simulink model "Pulse_Radar"  (R2026a)
settings: Solver=FixedStepDiscrete  StopTime=T_stop
values from neighbouring files (symbols this model uses):
  alpha = N_train * (Pfa^(-1/N_train) - 1)    (= 13.9867223149)    [centroid_2d.m]    (also in init.m = 17.2776488339)
  cfar_delay = (N_train/2) + (N_guard/2)    (= 116)    [init.m]
  cfar_window = [ones(1, N_train/2), zeros(1, N_guard + 1), ones(1, N_train/2)] / N_train    [init.m]
  current_seed = randi(100000)    [centroid_test.m]    (also in multi_target_test.m; os_cfar_test.m = seeds(k); run_monte_carlo.m; velocity_test.m = 12345)
  doppler_window = hamming(N_cpi)'    [init.m]
  drop_threshold_delay = 8    [init.m]
  fd = (2 * target_velocity) / lambda    [init.m]    (also in velocity_test.m)
  H_delay = exp(-1j*2*pi*k_idx*N_delay/N)    [init.m]
  hardware_delay_samples = matched_filter_delay + cfar_delay + drop_threshold_delay    [init.m]
  lambda = c / fc    (= 0.03)    [init.m]
  MTI_delay = N_PRI    [init.m]
  N_cpi = 16    [init.m]
  N_PRI = round(PRI / Ts)    [init.m]
  N_tau_p = round(tau_p / Ts)    [init.m]
  noise_variance_IQ = Pn / 2    (= 3.99251989225e-15)    [init.m]
  radar_const = (Pt * G^2 * lambda^2) ./ (((4*pi)^3) * (range.^4) * L)    [init.m]
  range = [20e3 40e3 70e3]    [init.m]
  range_per_sample = (c * Ts) / 2    (= 150)    [init.m]
  T_stop = N_cpi * PRI    (= 0.016)    [init.m]
  target_rcs = [1 1 1]    [init.m]
  Ts = 1e-6    (= 1e-06)    [init.m]
undefined symbols (not defined in the file or in its folder): dspblkCoreblockFVToolHelper, gcbh, get, jet, magnitude, Radix
libraries: dspxfrm3 x3, dspobslib x2, simulink x1
settings Model: Creator=daksh  LastModifiedBy=daksh

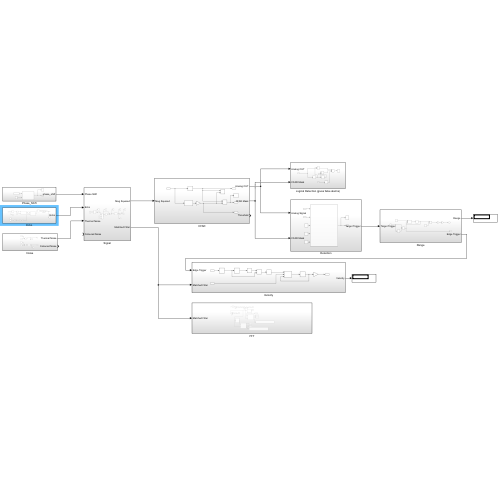
[thumbnail: Simulink's stored preview of the top-level diagram]
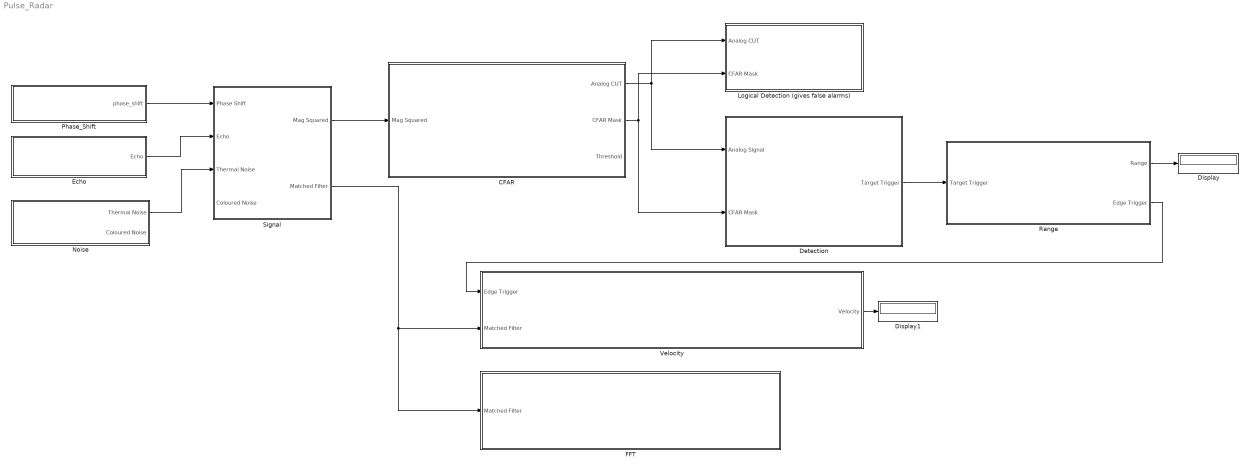
== system Pulse_Radar ==
  CFAR : Subsystem
  Detection : Subsystem
  Display : Display
  Display1 : Display
  Echo : Subsystem
  FFT : Subsystem
  Logical Detection (gives false alarms) : Subsystem
  Noise : Subsystem
  Phase_Shift : Subsystem
  Range : Subsystem
  Signal : Subsystem
  Velocity : Subsystem
  wires:
  Range/1(Range) -> Display/1
  Velocity/1(Velocity) -> Display1/1
  Noise/1(Thermal Noise) -> Signal/3(Thermal Noise)
  CFAR/1(Analog CUT) -> Logical Detection (gives false alarms)/1(Analog CUT), Detection/1(Analog Signal)
  CFAR/2(CFAR Mask) -> Detection/2(CFAR Mask), Logical Detection (gives false alarms)/2(CFAR Mask)
  Detection/1(Target Trigger) -> Range/1(Target Trigger)
  Range/2(Edge Trigger) -> Velocity/1(Edge Trigger)
  Echo/1(Echo) -> Signal/2(Echo)
  Phase_Shift/1(phase_shift) -> Signal/1(Phase Shift)
  Signal/1(Mag Squared) -> CFAR/1(Mag Squared)
  Signal/2(Matched Filter) -> FFT/1(Matched Filter), Velocity/2(Matched Filter)

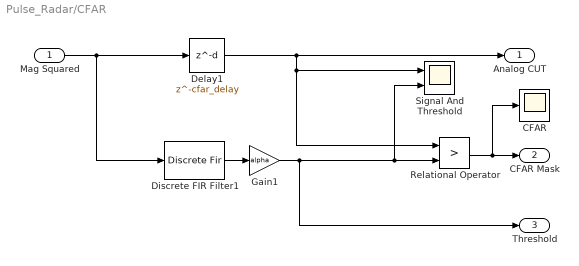
== system Pulse_Radar/CFAR ==
  Mag Squared : Inport
  CFAR : Scope
      settings: ActiveDisplayYMinimum=-1  ActiveDisplayYMaximum=1  DataLoggingVariableName=ScopeData10
  Delay1 : Delay  DelayLength=cfar_delay
  Discrete FIR Filter1 : DiscreteFir  LoadFcn=dspblkCoreblockFVToolHelper(gcbh,'load');  Coefficients=cfar_window
      settings: CopyFcn=dspblkCoreblockFVToolHelper(gcbh,'copy');  DeleteFcn=dspblkCoreblockFVToolHelper(gcbh,'close');  ModelCloseFcn=dspblkCoreblockFVToolHelper(gcbh,'close');  PreSaveFcn=dspblkCoreblockFVToolHelper(gcbh,'presave');  PostSaveFcn=dspblkCoreblockFVToolHelper(gcbh,'postsave');  CloseFcn=dspblkCoreblockFVToolHelper(gcbh,'close');
  Gain1 : Gain  Gain=alpha
  Relational Operator : RelationalOperator  Operator=>  OutDataTypeStr=boolean  RndMeth=Simplest  InputSameDT=off
  Signal And Threshold : Scope  NumInputPorts=2
      settings: ActiveDisplayYMinimum=-3.5614234572885921E-9  ActiveDisplayYMaximum=3.2052811115597338E-8  DataLoggingVariableName=ScopeData9
  Analog CUT : Outport
  CFAR Mask : Outport  Port=2
  Threshold : Outport  Port=3
  wires:
  Gain1/1 -> Signal And Threshold/2, Relational Operator/2, Threshold/1
  Discrete FIR Filter1/1 -> Gain1/1
  Mag Squared/1 -> Discrete FIR Filter1/1, Delay1/1
  Relational Operator/1 -> CFAR/1, CFAR Mask/1
  Delay1/1 -> Relational Operator/1, Signal And Threshold/1, Analog CUT/1

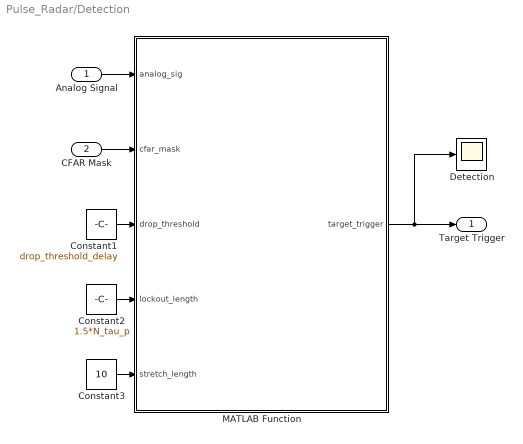
== system Pulse_Radar/Detection ==
  Analog Signal : Inport
  CFAR Mask : Inport  Port=2
  Constant1 : Constant  Value=drop_threshold_delay
  Constant2 : Constant  Value=1.5*N_tau_p
  Constant3 : Constant  Value=10
  Detection : Scope
      settings: ActiveDisplayYMinimum=-1  ActiveDisplayYMaximum=1  DataLoggingVariableName=ScopeData9
  MATLAB Function : MATLAB Function  TreatAsAtomicUnit=on
  Target Trigger : Outport
  wires:
  Constant3/1 -> MATLAB Function/5(stretch_length)
  Constant1/1 -> MATLAB Function/3(drop_threshold)
  Constant2/1 -> MATLAB Function/4(lockout_length)
  Analog Signal/1 -> MATLAB Function/1(analog_sig)
  CFAR Mask/1 -> MATLAB Function/2(cfar_mask)
  MATLAB Function/1(target_trigger) -> Detection/1, Target Trigger/1

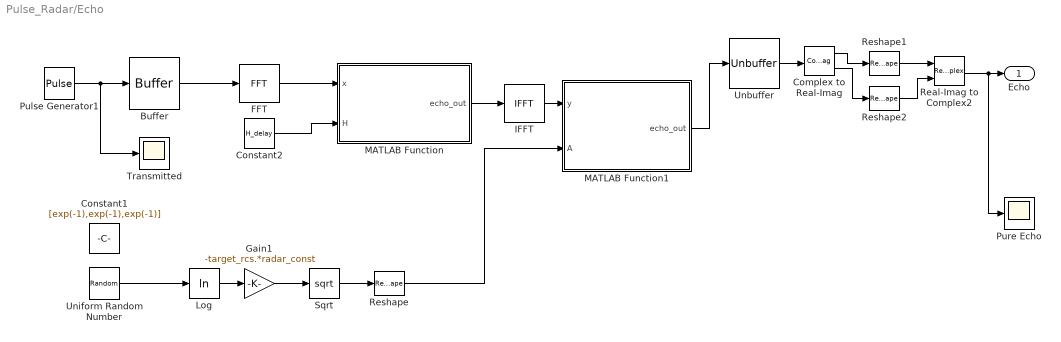
== system Pulse_Radar/Echo ==
  Buffer : Buffer  N=N_PRI  OutputFrames=off
  Complex to Real-Imag : ComplexToRealImag
  Constant1 : Constant  Value=[exp(-1),exp(-1),exp(-1)]
  Constant2 : Constant  Value=H_delay
  FFT : dspxfrm3/FFT  FFTImplementation=Auto  CompMethod=Table lookup  TableOpt=NEW  TableOptActive=Speed  BitRevOrder=off  Normalize=off  InheritFFTLength=on  FFTLength=64  WrapInput=on  roundingMode=Ceiling  overflowMode=off  firstCoeffDataTypeStr=Inherit: Same word length as input  firstCoeffLastDataTypeStr=Inherit: Same word length as input  outputMin=[]  outputMax=[]
  Gain1 : Gain  Gain=-target_rcs.*radar_const
  IFFT : dspxfrm3/IFFT  FFTImplementation=Auto  CompMethod=Table lookup  TableOpt=NEW  TableOptActive=Speed  BitRevOrder=off  cs_in=off  Normalize=on  InheritFFTLength=on  FFTLength=64  WrapInput=on  mode=Real  outSamplingMode=Sample based  roundingMode=Ceiling  overflowMode=off  firstCoeffDataTypeStr=Inherit: Same word length as input  firstCoeffLastDataTypeStr=Inherit: Same word length as input  outputMin=[]  outputMax=[]
  Log : Math  Operator=log
  MATLAB Function : MATLAB Function  TreatAsAtomicUnit=on
  MATLAB Function1 : MATLAB Function  TreatAsAtomicUnit=on
  Pulse Generator1 : DiscretePulseGenerator  Period=N_PRI  PulseWidth=N_tau_p  SampleTime=Ts
  Pure Echo : Scope
      settings: ActiveDisplayYMinimum=-1.2292527863379433E-7  ActiveDisplayYMaximum=1.1063275077038461E-6  DataLoggingVariableName=ScopeData2
  Real-Imag to Complex2 : RealImagToComplex
  Reshape : Reshape  OutputDimensionality=Customize  OutputDimensions=[1,numel(range)]
  Reshape1 : Reshape  OutputDimensionality=Customize  OutputDimensions=[numel(range), 1]
  Reshape2 : Reshape  OutputDimensionality=Customize  OutputDimensions=[numel(range), 1]
  Sqrt : Sqrt
  Transmitted : Scope
      settings: ActiveDisplayYMinimum=-1  ActiveDisplayYMaximum=1  DataLoggingVariableName=ScopeData3
  Unbuffer : Unbuffer
  Uniform Random Number : UniformRandomNumber  Minimum=0.0001*ones(1, numel(range))  Maximum=ones(size(range))  Seed=current_seed + 100*(1:numel(range))  SampleTime=T_stop
  Echo : Outport
  wires:
  Real-Imag to Complex2/1 -> Pure Echo/1, Echo/1
  Log/1 -> Gain1/1
  Gain1/1 -> Sqrt/1
  Sqrt/1 -> Reshape/1
  Uniform Random Number/1 -> Log/1
  Pulse Generator1/1 -> Transmitted/1, Buffer/1
  FFT/1 -> MATLAB Function/1(x)
  Buffer/1 -> FFT/1
  Constant2/1 -> MATLAB Function/2(H)
  MATLAB Function/1(echo_out) -> IFFT/1
  IFFT/1 -> MATLAB Function1/1(y)
  Reshape/1 -> MATLAB Function1/2(A)
  MATLAB Function1/1(echo_out) -> Unbuffer/1
  Reshape1/1 -> Real-Imag to Complex2/1
  Unbuffer/1 -> Complex to Real-Imag/1
  Complex to Real-Imag/1 -> Reshape1/1
  Complex to Real-Imag/2 -> Reshape2/1
  Reshape2/1 -> Real-Imag to Complex2/2

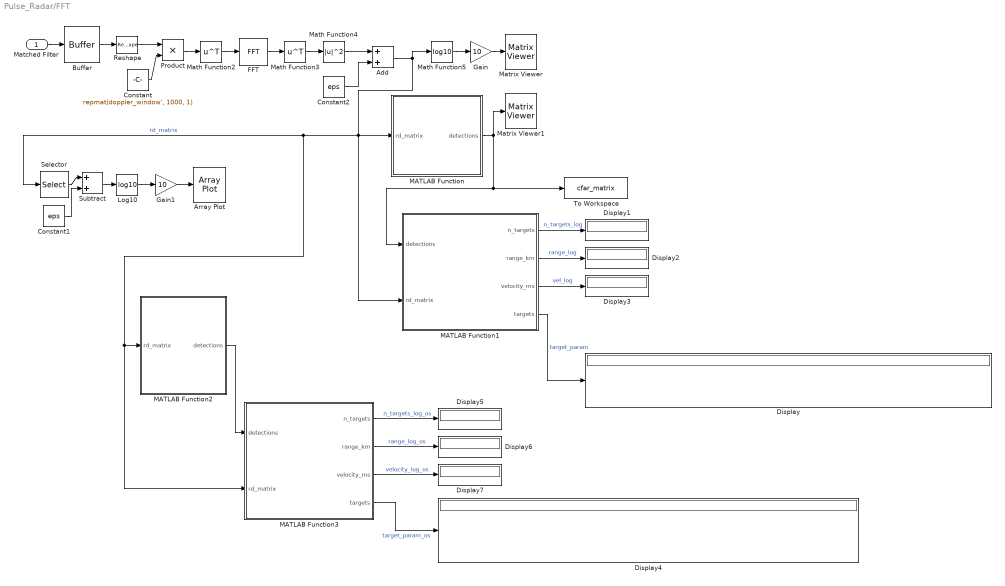
== system Pulse_Radar/FFT ==
  Matched Filter : Inport
  Add : Sum
  Array Plot : ArrayPlot  WindowPosition=[473.000000,199.000000,800.000000,500.000000,]  Visible=on  ScopeFrameLocation=window  YLimits=[-163.0987 -65.0075]
  Buffer : Buffer  N=N_PRI*N_cpi  OutputFrames=off
  Constant : Constant  Value=repmat(doppler_window', 1000, 1)  VectorParams1D=off
  Constant1 : Constant  Value=eps
  Constant2 : Constant  Value=eps
  Display{,1..7} (8 alike) : Display
  FFT : dspxfrm3/FFT  FFTImplementation=Radix-2  CompMethod=Table lookup  TableOpt=NEW  TableOptActive=Speed  BitRevOrder=off  Normalize=off  InheritFFTLength=on  FFTLength=64  WrapInput=on  roundingMode=Ceiling  overflowMode=off  firstCoeffDataTypeStr=Inherit: Same word length as input  firstCoeffLastDataTypeStr=Inherit: Same word length as input  outputMin=[]  outputMax=[]
  Gain : Gain  Gain=10
  Gain1 : Gain  Gain=10
  Log10 : Math  Operator=log10
  MATLAB Function : MATLAB Function  TreatAsAtomicUnit=on
  MATLAB Function1 : MATLAB Function  TreatAsAtomicUnit=on
  MATLAB Function2 : MATLAB Function  TreatAsAtomicUnit=on
  MATLAB Function3 : MATLAB Function  TreatAsAtomicUnit=on
  Math Function2 : Math  Operator=transpose
  Math Function3 : Math  Operator=transpose
  Math Function4 : Math  Operator=magnitude^2
  Math Function5 : Math  Operator=log10
  Matrix Viewer : dspobslib/Matrix Viewer  ImageParams=off  CMapStr=jet(256)  AxisColorbar=on  AxisParams=off  AxisOrigin=Upper left corner  AxisTickMode=Auto  XTickRange=[0 1]  YTickRange=[0 1]  XLabel=X-axis  YLabel=Y-axis  ZLabel=Z-axis  FigPos=get(0,'defaultfigureposition')  AxisZoom=off
      settings: YMin=-100  YMax=0
  Matrix Viewer1 : dspobslib/Matrix Viewer  ImageParams=off  CMapStr=gray  AxisColorbar=on  AxisParams=off  AxisOrigin=Upper left corner  AxisTickMode=Auto  XTickRange=[0 1]  YTickRange=[0 1]  XLabel=X-axis  YLabel=Y-axis  ZLabel=Z-axis  FigPos=get(0,'defaultfigureposition')  AxisZoom=off
      settings: YMin=0  YMax=1
  Product : Product
  Reshape : Reshape  OutputDimensionality=Customize  OutputDimensions=[N_PRI, N_cpi]
  Selector : Selector  NumberOfDimensions=2  InputPortWidth=3  IndexOptions=Select all,Select all  Indices=[1 3],1  OutputSizes=1,1
  Subtract : Sum
  To Workspace : ToWorkspace  VariableName=cfar_matrix  SampleTime=-1
  wires:
  Math Function5/1 -> Gain/1
  Math Function3/1 -> Math Function4/1
  FFT/1 -> Math Function3/1
  Gain/1 -> Matrix Viewer/1
  Math Function2/1 -> FFT/1
  Buffer/1 -> Reshape/1
  Matched Filter/1 -> Buffer/1
  MATLAB Function/1(detections) -> Matrix Viewer1/1, MATLAB Function1/1(detections), To Workspace/1
  Reshape/1 -> Product/1
  Constant/1 -> Product/2
  Product/1 -> Math Function2/1
  Log10/1 -> Gain1/1
  Gain1/1 -> Array Plot/1
  Subtract/1 -> Log10/1
  Selector/1 -> Subtract/1
  Constant1/1 -> Subtract/2
  Math Function4/1 -> Add/1
  Add/1 -> MATLAB Function1/2(rd_matrix), MATLAB Function/1(rd_matrix), MATLAB Function3/2(rd_matrix), MATLAB Function2/1(rd_matrix), Selector/1, Math Function5/1  "rd_matrix"
  Constant2/1 -> Add/2
  MATLAB Function1/4(targets) -> Display/1  "target_param"
  MATLAB Function1/1(n_targets) -> Display1/1  "n_targets_log"
  MATLAB Function1/2(range_km) -> Display2/1  "range_log"
  MATLAB Function1/3(velocity_ms) -> Display3/1  "vel_log"
  MATLAB Function2/1(detections) -> MATLAB Function3/1(detections)
  MATLAB Function3/4(targets) -> Display4/1  "target_param_os"
  MATLAB Function3/1(n_targets) -> Display5/1  "n_targets_log_os"
  MATLAB Function3/2(range_km) -> Display6/1  "range_log_os"
  MATLAB Function3/3(velocity_ms) -> Display7/1  "velocity_log_os"

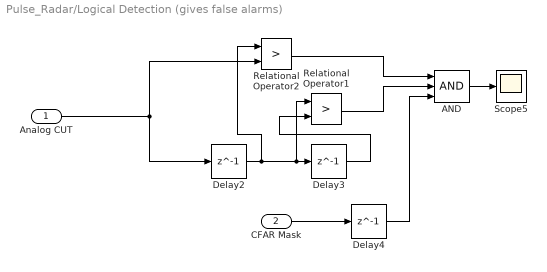
== system Pulse_Radar/Logical Detection (gives false alarms) ==
  Analog CUT : Inport
  CFAR Mask : Inport  Port=2
  AND : Logic  Inputs=3  IconShape=distinctive  AllPortsSameDT=off  OutDataTypeStr=boolean
  Delay2 : Delay  DelayLength=1
  Delay3 : Delay  DelayLength=1
  Delay4 : Delay  DelayLength=1
  Relational Operator1 : RelationalOperator  Operator=>  OutDataTypeStr=boolean  RndMeth=Simplest  InputSameDT=off
  Relational Operator2 : RelationalOperator  Operator=>  OutDataTypeStr=boolean  RndMeth=Simplest  InputSameDT=off
  Scope5 : Scope
      settings: ActiveDisplayYMinimum=-0.12499999999999997  ActiveDisplayYMaximum=1.125  DataLoggingVariableName=ScopeData5
  wires:
  Relational Operator2/1 -> AND/1
  AND/1 -> Scope5/1
  Delay2/1 -> Relational Operator2/1, Relational Operator1/1, Delay3/1
  Delay3/1 -> Relational Operator1/2
  Relational Operator1/1 -> AND/2
  Delay4/1 -> AND/3
  Analog CUT/1 -> Delay2/1, Relational Operator2/2
  CFAR Mask/1 -> Delay4/1

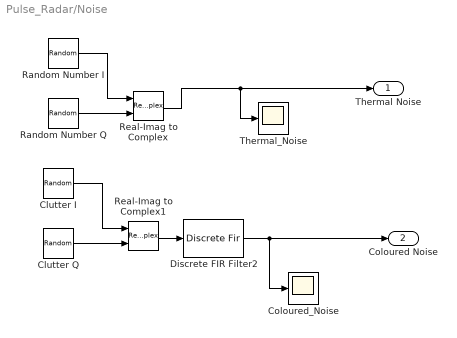
== system Pulse_Radar/Noise ==
  Clutter I : RandomNumber  Variance=noise_variance_IQ*50  Seed=current_seed+2  SampleTime=Ts
  Clutter Q : RandomNumber  Variance=noise_variance_IQ*50  Seed=current_seed+3  SampleTime=Ts
  Coloured_Noise : Scope
      settings: ActiveDisplayYMinimum=-1  ActiveDisplayYMaximum=1
  Discrete FIR Filter2 : DiscreteFir  LoadFcn=dspblkCoreblockFVToolHelper(gcbh,'load');  Coefficients=ones(1,100)/10
      settings: CopyFcn=dspblkCoreblockFVToolHelper(gcbh,'copy');  DeleteFcn=dspblkCoreblockFVToolHelper(gcbh,'close');  ModelCloseFcn=dspblkCoreblockFVToolHelper(gcbh,'close');  PreSaveFcn=dspblkCoreblockFVToolHelper(gcbh,'presave');  PostSaveFcn=dspblkCoreblockFVToolHelper(gcbh,'postsave');  CloseFcn=dspblkCoreblockFVToolHelper(gcbh,'close');
  Random Number I : RandomNumber  Variance=noise_variance_IQ  Seed=current_seed  SampleTime=Ts
  Random Number Q : RandomNumber  Variance=noise_variance_IQ  Seed=current_seed +1  SampleTime=Ts
  Real-Imag to Complex : RealImagToComplex
  Real-Imag to Complex1 : RealImagToComplex
  Thermal_Noise : Scope
      settings: ActiveDisplayYMinimum=-3.1205725347729866E-7  ActiveDisplayYMaximum=3.0716380696194773E-7
  Thermal Noise : Outport
  Coloured Noise : Outport  Port=2
  wires:
  Real-Imag to Complex/1 -> Thermal_Noise/1, Thermal Noise/1
  Random Number I/1 -> Real-Imag to Complex/1
  Random Number Q/1 -> Real-Imag to Complex/2
  Clutter I/1 -> Real-Imag to Complex1/1
  Clutter Q/1 -> Real-Imag to Complex1/2
  Real-Imag to Complex1/1 -> Discrete FIR Filter2/1
  Discrete FIR Filter2/1 -> Coloured_Noise/1, Coloured Noise/1

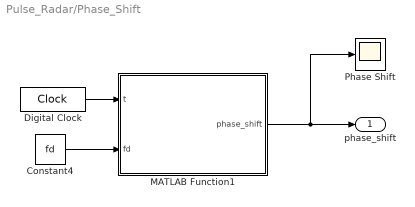
== system Pulse_Radar/Phase_Shift ==
  Constant4 : Constant  Value=fd
  Digital Clock : DigitalClock  SampleTime=Ts
  MATLAB Function1 : MATLAB Function  TreatAsAtomicUnit=on
  Phase Shift : Scope
      settings: ActiveDisplayYMinimum=-1.0804489386242251  ActiveDisplayYMaximum=1.1802346006807898  DataLoggingVariableName=ScopeData11
  phase_shift : Outport
  wires:
  Digital Clock/1 -> MATLAB Function1/1(t)
  Constant4/1 -> MATLAB Function1/2(fd)
  MATLAB Function1/1(phase_shift) -> Phase Shift/1, phase_shift/1

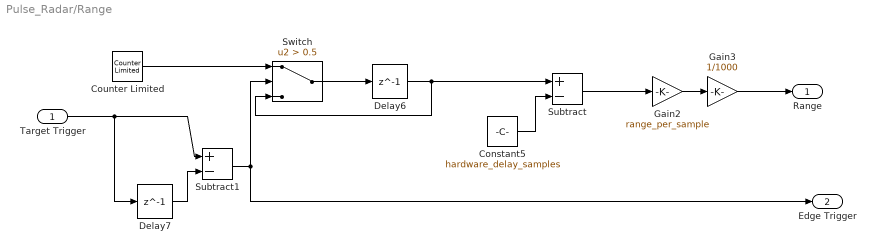
== system Pulse_Radar/Range ==
  Target Trigger : Inport
  Constant5 : Constant  Value=hardware_delay_samples
  Counter Limited : simulink/Sources/Counter Limited  uplimit=N_PRI-1  tsamp=Ts
  Delay6 : Delay  DelayLength=1
  Delay7 : Delay  DelayLength=1
  Gain2 : Gain  Gain=range_per_sample
  Gain3 : Gain  Gain=1/1000
  Subtract : Sum  Inputs=+-
  Subtract1 : Sum  Inputs=+-
  Switch : Switch  Criteria=u2 > Threshold  Threshold=0.5  SaturateOnIntegerOverflow=off  InputSameDT=off
  Range : Outport
  Edge Trigger : Outport  Port=2
  wires:
  Subtract1/1 -> Edge Trigger/1, Switch/2
  Delay7/1 -> Subtract1/2
  Subtract/1 -> Gain2/1
  Constant5/1 -> Subtract/2
  Delay6/1 -> Subtract/1, Switch/3
  Switch/1 -> Delay6/1
  Counter Limited/1 -> Switch/1
  Gain2/1 -> Gain3/1
  Target Trigger/1 -> Delay7/1, Subtract1/1
  Gain3/1 -> Range/1

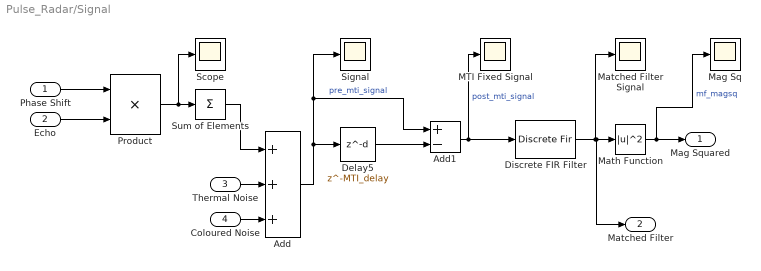
== system Pulse_Radar/Signal ==
  Phase Shift : Inport
  Echo : Inport  Port=2
  Thermal Noise : Inport  Port=3
  Coloured Noise : Inport  Port=4
  Add : Sum  Inputs=+++
  Add1 : Sum  Inputs=+-
  Delay5 : Delay  DelayLength=MTI_delay
  Discrete FIR Filter : DiscreteFir  LoadFcn=dspblkCoreblockFVToolHelper(gcbh,'load');  Coefficients=range_window'
      settings: CopyFcn=dspblkCoreblockFVToolHelper(gcbh,'copy');  DeleteFcn=dspblkCoreblockFVToolHelper(gcbh,'close');  ModelCloseFcn=dspblkCoreblockFVToolHelper(gcbh,'close');  PreSaveFcn=dspblkCoreblockFVToolHelper(gcbh,'presave');  PostSaveFcn=dspblkCoreblockFVToolHelper(gcbh,'postsave');  CloseFcn=dspblkCoreblockFVToolHelper(gcbh,'close');
  MTI Fixed Signal : Scope
      settings: ActiveDisplayYMinimum=-1  ActiveDisplayYMaximum=1  DataLoggingVariableName=ScopeData6
  Mag Sq : Scope
      settings: ActiveDisplayYMinimum=-3.4748663291483945E-10  ActiveDisplayYMaximum=3.1273800545095807E-9  DataLoggingVariableName=ScopeData8
  Matched Filter Signal : Scope
      settings: ActiveDisplayYMinimum=-5.85240966632453E-5  ActiveDisplayYMaximum=5.9924573113531178E-5  DataLoggingVariableName=ScopeData7
  Math Function : Math  Operator=magnitude^2
  Product : Product
  Scope : Scope
      settings: ActiveDisplayYMinimum=-1.2284656809866782E-6  ActiveDisplayYMaximum=1.2223896980187576E-6  DataLoggingVariableName=ScopeData12
  Signal : Scope
      settings: ActiveDisplayYMinimum=-1  ActiveDisplayYMaximum=1  DataLoggingVariableName=ScopeData4
  Sum of Elements : Sum  Inputs=+
  Mag Squared : Outport
  Matched Filter : Outport  Port=2
  wires:
  Add1/1 -> MTI Fixed Signal/1, Discrete FIR Filter/1  "post_mti_signal"
  Delay5/1 -> Add1/2
  Add/1 -> Signal/1, Add1/1, Delay5/1  "pre_mti_signal"
  Thermal Noise/1 -> Add/2
  Coloured Noise/1 -> Add/3
  Math Function/1 -> Mag Sq/1, Mag Squared/1  "mf_magsq"
  Discrete FIR Filter/1 -> Matched Filter Signal/1, Matched Filter/1, Math Function/1
  Echo/1 -> Product/2
  Phase Shift/1 -> Product/1
  Product/1 -> Scope/1, Sum of Elements/1
  Sum of Elements/1 -> Add/1

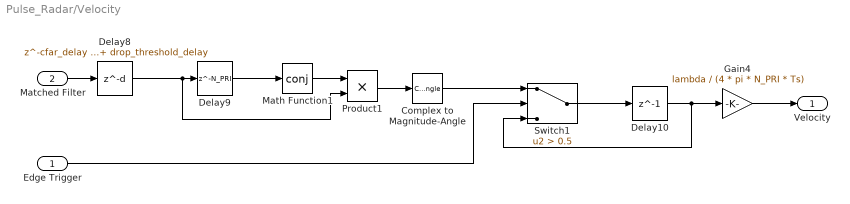
== system Pulse_Radar/Velocity ==
  Edge Trigger : Inport
  Matched Filter : Inport  Port=2
  Complex to Magnitude-Angle : ComplexToMagnitudeAngle  Output=Angle
  Delay10 : Delay  DelayLength=1
  Delay8 : Delay  DelayLength=cfar_delay + drop_threshold_delay
  Delay9 : Delay  DelayLength=N_PRI
  Gain4 : Gain  Gain=lambda / (4 * pi * N_PRI * Ts)
  Math Function1 : Math  Operator=conj
  Product1 : Product
  Switch1 : Switch  Criteria=u2 > Threshold  Threshold=0.5  SaturateOnIntegerOverflow=off  InputSameDT=off
  Velocity : Outport
  wires:
  Delay9/1 -> Math Function1/1
  Delay10/1 -> Gain4/1, Switch1/3
  Delay8/1 -> Product1/2, Delay9/1
  Product1/1 -> Complex to Magnitude-Angle/1
  Complex to Magnitude-Angle/1 -> Switch1/1
  Math Function1/1 -> Product1/1
  Switch1/1 -> Delay10/1
  Matched Filter/1 -> Delay8/1
  Gain4/1 -> Velocity/1
  Edge Trigger/1 -> Switch1/2

== matlab function Pulse_Radar/Phase_Shift/MATLAB Function1 ==
  data: t input; phase_shift output; fd input
function phase_shift = apply_doppler(t, fd)
    phase_shift = exp(1j * 2 * pi * fd * t);
end

== matlab function Pulse_Radar/FFT/MATLAB Function ==
  data: rd_matrix input; detections output
function detections = cfar_2d(rd_matrix)
% 2D cell-averaging CFAR on a range-Doppler power map.
% rd_matrix : 1000x16 LINEAR power (|u|^2), not dB
% detections: 1000x16 binary map
%
% Changes from the previous version:
%   1. Gr 200 -> 100 (half the 199-sample matched-filter triangle).
%   2. The matrix is padded, so EVERY range row is tested. Before, rows within
%      Tr+Gr of either end were skipped, which made close targets undetectable.
%   3. The Doppler axis is padded circularly (velocity wraps around).
% The same code runs in the Simulink MATLAB Function block and from a script.

    [num_ranges, num_dopplers] = size(rd_matrix);

    Pfa = 1e-6;
    Tr = 16;    Td = 1;     % training cells (range, Doppler), per side
    Gr = 100;   Gd = 3;     % guard cells    (range, Doppler), per side

    N_train = (2*(Tr+Gr)+1)*(2*(Td+Gd)+1) - (2*Gr+1)*(2*Gd+1);
    alpha   = N_train * (Pfa^(-1/N_train) - 1);

    pr = Tr + Gr;           % half-height of the window
    pd = Td + Gd;           % half-width  of the window

    % Pad with a noise-level value. For exponential noise power, median = mean*ln2,
    % so median/ln2 estimates the mean and is not pulled up by the target.
    % Zeros would make the edge estimate too low and cause false alarms there.
    noise_level = median(rd_matrix(:)) / log(2);
    rd_pad = noise_level * ones(num_ranges + 2*pr, num_dopplers + 2*pd);
    rd_pad(pr+1:pr+num_ranges, pd+1:pd+num_dopplers) = rd_matrix;
    rd_pad(pr+1:pr+num_ranges, 1:pd) = rd_matrix(:, num_dopplers-pd+1:num_dopplers);
    rd_pad(pr+1:pr+num_ranges, pd+num_dopplers+1:end) = rd_matrix(:, 1:pd);

    detections = zeros(num_ranges, num_dopplers);

    for r = 1:num_ranges
        for d = 1:num_dopplers
            rc = r + pr;                                   % cell position in padded matrix
            dc = d + pd;

            window = rd_pad(rc-pr : rc+pr, dc-pd : dc+pd); % outer window
            guard  = rd_pad(rc-Gr : rc+Gr, dc-Gd : dc+Gd); % guard region + CUT

            noise_avg = (sum(window(:)) - sum(guard(:))) / N_train;

            if rd_pad(rc, dc) > alpha * noise_avg
                detections(r, d) = 1;
            end
        end
    end
end

== matlab function Pulse_Radar/Detection/MATLAB Function ==
  data: analog_sig input; target_trigger output; cfar_mask input; drop_threshold input; lockout_length input; stretch_length input
function target_trigger = extract_plot(analog_sig, cfar_mask, drop_threshold, lockout_length, stretch_length)
    % persistent memory registers
    persistent drop_counter lockout_timer last_sig display_timer;
    
    if isempty(drop_counter)
        drop_counter = 0;
        lockout_timer = 0;
        last_sig = 0;
        display_timer = 0;
    end
    
    target_trigger = 0;
    
    % 1. Scope Stretcher (Visual)
    if display_timer > 0
        target_trigger = 1;
        display_timer = display_timer - 1;
    end
    
    % 2. Advance Lockout
    if lockout_timer > 0
        lockout_timer = lockout_timer - 1;
    end
    
    % 3. Peak Detection Logic
    if cfar_mask == 1 && lockout_timer == 0
        
        if analog_sig < last_sig
            drop_counter = drop_counter + 1;
        else
            drop_counter = 0; % Reset on any rise
        end
        
        % The hardcoded 5 is now dynamically controlled by drop_threshold
        if drop_counter == drop_threshold
            target_trigger = 1;      
            display_timer = stretch_length;      
            lockout_timer = lockout_length;     
            drop_counter = 0;        
        end
        
    else
        drop_counter = 0;
    end
    
    last_sig = analog_sig;
end

== matlab function Pulse_Radar/FFT/MATLAB Function1 ==
  data: detections input; n_targets output; range_km output; velocity_ms output; rd_matrix input; targets output
function [n_targets, range_km, velocity_ms, targets] = centroid_2d(detections, rd_matrix)
% Group CFAR detections into clusters and report one target per cluster.
% Written to run both from a script and inside a Simulink MATLAB Function block:
% fixed-size outputs, plain loops, no toolbox calls.
%
% rd_matrix  : 1000x16 linear power
% detections : 1000x16 binary map from cfar_2d
% targets    : 8x8, one row per cluster (unused rows are zero):
%   [peak_row, peak_col, centroid_row, centroid_col, total_power, n_cells, range_m, velocity_ms]
% n_targets  : number of valid rows (at most MAXT)
% range_km    : range of the STRONGEST cluster, in km  (NaN if nothing was detected)
% velocity_ms : velocity of the STRONGEST cluster, m/s (NaN if nothing was detected)
%
% Range comes from the PEAK row (150 m bins already resolve it).
% Velocity comes from the CENTROID column (0.94 m/s bins are coarse).
% Clusters are joined across the Doppler wrap-around (column 16 touches column 1).

    MAXT         = 8;
    RANGE_OFFSET = 100;        % rows; peak row = N_delay + 100 for a target at delay N_delay
    RANGE_PER_ROW = 150;       % m, c*Ts/2          (keep in step with init.m)
    VEL_PER_BIN   = 0.9375;    % m/s, lambda/(2*N_cpi*PRI)

    [nr, nd] = size(detections);
    targets     = zeros(MAXT, 8);
    n_targets   = 0;
    range_km    = NaN;
    velocity_ms = NaN;

    visited = false(nr, nd);
    stack_r = zeros(nr*nd, 1);
    stack_d = zeros(nr*nd, 1);
    cell_r  = zeros(nr*nd, 1);
    cell_d  = zeros(nr*nd, 1);

    for r0 = 1:nr
        for d0 = 1:nd
            if detections(r0, d0) ~= 0 && ~visited(r0, d0)

                % ---- flood fill (8-connected, circular in Doppler) ----
                sp = 1;  stack_r(1) = r0;  stack_d(1) = d0;
                visited(r0, d0) = true;
                nc = 0;
                while sp > 0
                    r = stack_r(sp);  d = stack_d(sp);  sp = sp - 1;
                    nc = nc + 1;  cell_r(nc) = r;  cell_d(nc) = d;
                    for dr = -1:1
                        for dj = -1:1
                            if dr == 0 && dj == 0
                                continue;
                            end
                            rr = r + dr;
                            if rr < 1 || rr > nr
                                continue;
                            end
                            dd = mod(d - 1 + dj, nd) + 1;
                            if detections(rr, dd) ~= 0 && ~visited(rr, dd)
                                visited(rr, dd) = true;
                                sp = sp + 1;
                                stack_r(sp) = rr;  stack_d(sp) = dd;
                            end
                        end
                    end
                end

                % ---- peak cell of the cluster ----
                pmax = -1;  pr = 0;  pc = 0;
                for i = 1:nc
                    p = rd_matrix(cell_r(i), cell_d(i));
                    if p > pmax
                        pmax = p;  pr = cell_r(i);  pc = cell_d(i);
                    end
                end

                % ---- power-weighted centroid (columns measured as an offset from the peak, so wrap-around is safe) ----
                P = 0;  Sr = 0;  Sc = 0;
                for i = 1:nc
                    p   = rd_matrix(cell_r(i), cell_d(i));
                    off = mod(cell_d(i) - pc + nd/2, nd) - nd/2;
                    P   = P  + p;
                    Sr  = Sr + cell_r(i) * p;
                    Sc  = Sc + off * p;
                end
                cen_r = Sr / P;
                cen_c = mod(pc + Sc/P - 1, nd) + 1;

                % ---- physical units ----
                b = cen_c - 1;                 % Doppler bin, 0..nd-1
                if b > nd/2
                    b = b - nd;                % upper half of the bins = negative velocity
                end

                if n_targets < MAXT
                    n_targets = n_targets + 1;
                    targets(n_targets, :) = [pr, pc, cen_r, cen_c, P, nc, ...
                                             (pr - RANGE_OFFSET) * RANGE_PER_ROW, ...
                                             b * VEL_PER_BIN];
                end
            end
        end
    end

    % ---- headline numbers: the strongest cluster (highest total power) ----
    best = 0;  best_power = -1;
    for i = 1:n_targets
        if targets(i, 5) > best_power
            best_power = targets(i, 5);
            best = i;
        end
    end
    if best > 0
        range_km    = targets(best, 7) / 1000;
        velocity_ms = targets(best, 8);
    end
end

== matlab function Pulse_Radar/Echo/MATLAB Function ==
  data: x input; echo_out output; H input
function echo_out = apply_H(x, H)
    echo_out = x .* H;    % 1000x1 .* 1000x3, broadcasts correctly in MATLAB code
end

== matlab function Pulse_Radar/Echo/MATLAB Function1 ==
  data: y input; echo_out output; A input
function echo_out = apply_amplitude(y, A)
% y : 1000x3, complex time-domain signal from IFFT
% A : 3x1 or 1x3, random amplitude per target
% echo_out : 1000x3, complex

    N = size(y, 2);
    A = reshape(A, 1, N);
    echo_out = y .* A;
end

== matlab function Pulse_Radar/FFT/MATLAB Function2 ==
  data: rd_matrix input; detections output
function detections = os_cfar_2d(rd_matrix)
% 2D Order-Statistic CFAR. Same guard/training geometry as cfar_2d, but
% instead of averaging all training cells, sorts them and uses the k-th
% smallest as the noise estimate. A strong interferer only contaminates
% part of the training window, so a percentile below that fraction ignores
% it -- this is the fix for a strong target masking a weaker nearby one.

    [num_ranges, num_dopplers] = size(rd_matrix);

    Pfa    = 1e-6;
    Tr = 16;   Td = 1;      % training cells (range, Doppler), per side
    Gr = 100;  Gd = 2;      % guard cells    (range, Doppler), per side
    k_frac = 0.75;          % use the 75th-percentile training cell

    pr = Tr + Gr;
    pd = Td + Gd;

    N_train = (2*(Tr+Gr)+1)*(2*(Td+Gd)+1) - (2*Gr+1)*(2*Gd+1);
    k = max(1, round(k_frac * N_train));
    alpha = k * (Pfa^(-1/k) - 1);

    % Pad the same way as cfar_2d: noise-level value in range, circular in Doppler
    noise_level = median(rd_matrix(:)) / log(2);
    rd_pad = noise_level * ones(num_ranges + 2*pr, num_dopplers + 2*pd);
    rd_pad(pr+1:pr+num_ranges, pd+1:pd+num_dopplers) = rd_matrix;
    rd_pad(pr+1:pr+num_ranges, 1:pd) = rd_matrix(:, num_dopplers-pd+1:num_dopplers);
    rd_pad(pr+1:pr+num_ranges, pd+num_dopplers+1:end) = rd_matrix(:, 1:pd);

    % Precompute training-cell offsets (outer window minus guard box)
    n_off = 0;
    off_r = zeros((2*pr+1)*(2*pd+1), 1);
    off_c = zeros((2*pr+1)*(2*pd+1), 1);
    for dr = -pr:pr
        for dc = -pd:pd
            if abs(dr) > Gr || abs(dc) > Gd
                n_off = n_off + 1;
                off_r(n_off) = dr;
                off_c(n_off) = dc;
            end
        end
    end

    detections = zeros(num_ranges, num_dopplers);
    train_vals = zeros(N_train, 1);

    for r = 1:num_ranges
        for d = 1:num_dopplers
            rc = r + pr;
            dc = d + pd;
            for i = 1:N_train
                train_vals(i) = rd_pad(rc + off_r(i), dc + off_c(i));
            end
            sorted_vals = sort(train_vals);
            noise_est   = sorted_vals(k);
            if rd_pad(rc, dc) > alpha * noise_est
                detections(r, d) = 1;
            end
        end
    end
end

== matlab function Pulse_Radar/FFT/MATLAB Function3 ==
  data: detections input; n_targets output; range_km output; velocity_ms output; rd_matrix input; targets output
function [n_targets, range_km, velocity_ms, targets] = centroid_2d(detections, rd_matrix)
% Group CFAR detections into clusters and report one target per cluster.
% Written to run both from a script and inside a Simulink MATLAB Function block:
% fixed-size outputs, plain loops, no toolbox calls.
%
% rd_matrix  : 1000x16 linear power
% detections : 1000x16 binary map from cfar_2d
% targets    : 8x8, one row per cluster (unused rows are zero):
%   [peak_row, peak_col, centroid_row, centroid_col, total_power, n_cells, range_m, velocity_ms]
% n_targets  : number of valid rows (at most MAXT)
% range_km    : range of the STRONGEST cluster, in km  (NaN if nothing was detected)
% velocity_ms : velocity of the STRONGEST cluster, m/s (NaN if nothing was detected)
%
% Range comes from the PEAK row (150 m bins already resolve it).
% Velocity comes from the CENTROID column (0.94 m/s bins are coarse).
% Clusters are joined across the Doppler wrap-around (column 16 touches column 1).

    MAXT         = 8;
    RANGE_OFFSET = 100;        % rows; peak row = N_delay + 100 for a target at delay N_delay
    RANGE_PER_ROW = 150;       % m, c*Ts/2          (keep in step with init.m)
    VEL_PER_BIN   = 0.9375;    % m/s, lambda/(2*N_cpi*PRI)

    [nr, nd] = size(detections);
    targets     = zeros(MAXT, 8);
    n_targets   = 0;
    range_km    = NaN;
    velocity_ms = NaN;

    visited = false(nr, nd);
    stack_r = zeros(nr*nd, 1);
    stack_d = zeros(nr*nd, 1);
    cell_r  = zeros(nr*nd, 1);
    cell_d  = zeros(nr*nd, 1);

    for r0 = 1:nr
        for d0 = 1:nd
            if detections(r0, d0) ~= 0 && ~visited(r0, d0)

                % ---- flood fill (8-connected, circular in Doppler) ----
                sp = 1;  stack_r(1) = r0;  stack_d(1) = d0;
                visited(r0, d0) = true;
                nc = 0;
                while sp > 0
                    r = stack_r(sp);  d = stack_d(sp);  sp = sp - 1;
                    nc = nc + 1;  cell_r(nc) = r;  cell_d(nc) = d;
                    for dr = -1:1
                        for dj = -1:1
                            if dr == 0 && dj == 0
                                continue;
                            end
                            rr = r + dr;
                            if rr < 1 || rr > nr
                                continue;
                            end
                            dd = mod(d - 1 + dj, nd) + 1;
                            if detections(rr, dd) ~= 0 && ~visited(rr, dd)
                                visited(rr, dd) = true;
                                sp = sp + 1;
                                stack_r(sp) = rr;  stack_d(sp) = dd;
                            end
                        end
                    end
                end

                % ---- peak cell of the cluster ----
                pmax = -1;  pr = 0;  pc = 0;
                for i = 1:nc
                    p = rd_matrix(cell_r(i), cell_d(i));
                    if p > pmax
                        pmax = p;  pr = cell_r(i);  pc = cell_d(i);
                    end
                end

                % ---- power-weighted centroid (columns measured as an offset from the peak, so wrap-around is safe) ----
                P = 0;  Sr = 0;  Sc = 0;
                for i = 1:nc
                    p   = rd_matrix(cell_r(i), cell_d(i));
                    off = mod(cell_d(i) - pc + nd/2, nd) - nd/2;
                    P   = P  + p;
                    Sr  = Sr + cell_r(i) * p;
                    Sc  = Sc + off * p;
                end
                cen_r = Sr / P;
                cen_c = mod(pc + Sc/P - 1, nd) + 1;

                % ---- physical units ----
                b = cen_c - 1;                 % Doppler bin, 0..nd-1
                if b > nd/2
                    b = b - nd;                % upper half of the bins = negative velocity
                end

                if n_targets < MAXT
                    n_targets = n_targets + 1;
                    targets(n_targets, :) = [pr, pc, cen_r, cen_c, P, nc, ...
                                             (pr - RANGE_OFFSET) * RANGE_PER_ROW, ...
                                             b * VEL_PER_BIN];
                end
            end
        end
    end

    % ---- headline numbers: the strongest cluster (highest total power) ----
    best = 0;  best_power = -1;
    for i = 1:n_targets
        if targets(i, 5) > best_power
            best_power = targets(i, 5);
            best = i;
        end
    end
    if best > 0
        range_km    = targets(best, 7) / 1000;
        velocity_ms = targets(best, 8);
    end
end
